simulink model "OCC_DQ_RCC_PO_BOOST_COMMON_GROUND_UPM"  (R2023a)
settings: Solver=ode1  StartTime=0.0  StopTime=5  FixedStep=1e-6  MaxStep=1e-6  RelTol=1e-3  EnableMultiTasking=on
undefined symbols (not defined in the file or in its folder): DiscIntNeverNeededParam
libraries: simulink x15, spsSeriesRLCBranchLib x14, spsVoltageMeasurementLib x8, slpidlib x7, spsDiodeLib x6, spsFirstOrderFilterLib x6, spsMosfetLib x5, powerlib_extras x5, spsCurrentMeasurementLib x4, spsAlphaBetaZerotodq0Lib x3, eePowerMeasurement x2, spsACVoltageSourceLib x1
(part 2 of 2)

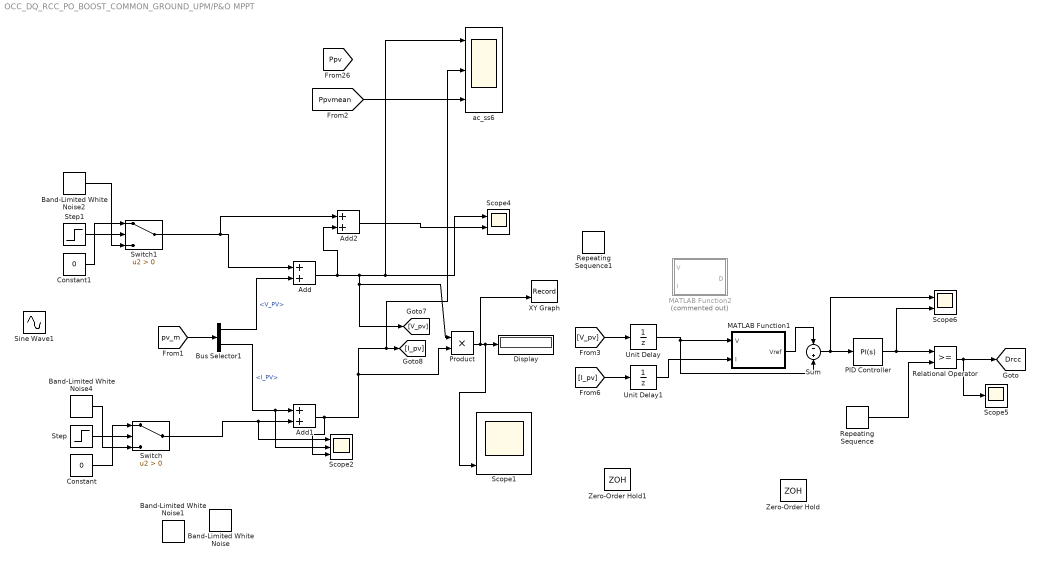
== system OCC_DQ_RCC_PO_BOOST_COMMON_GROUND_UPM/P&O MPPT  ==
  Add : Sum
  Add1 : Sum
  Add2 : Sum
  Band-Limited White Noise : simulink/Sources/Band-Limited White Noise  Cov=[1.74e-6]  Ts=1e-6  seed=[23341]
  Band-Limited White Noise1 : simulink/Sources/Band-Limited White Noise  Cov=[5.776e-9]  Ts=1e-6  seed=[23341]
  Band-Limited White Noise2 : simulink/Sources/Band-Limited White Noise  Cov=[6.6e-7]  Ts=1e-6  seed=[23341]
  Band-Limited White Noise4 : simulink/Sources/Band-Limited White Noise  Cov=[3.58e-10]  Ts=1e-6  seed=[23341]
  Bus Selector1 : BusSelector  OutputSignals=V_PV,I_PV
  Constant : Constant  Value=0
  Constant1 : Constant  Value=0
  Display : Display
  MATLAB Function1 : MATLAB Function  TreatAsAtomicUnit=on
  MATLAB Function2 : MATLAB Function  Commented=on  TreatAsAtomicUnit=on
  PID Controller : slpidlib/PID Controller  Controller=PI  Form=Parallel  TimeDomain=Continuous-time  UseExternalTs=off  SampleTime=-1  IntegratorMethod=Forward Euler  FilterMethod=Forward Euler  ControllerParametersSource=internal  P=0.011  I=15  UseKiTs=off  D=0  N=100  UseFilter=on  TunerSelectOption=Transfer Function Based (PID Tuner App)  InitialConditionSource=internal  InitialConditionForIntegrator=0  InitialConditionForFilter=0  DifferentiatorICPrevScaledInput=0  ExternalReset=none  TrackingMode=off  Kt=1  LimitOutput=on  SatLimitsSource=internal  UpperSaturationLimit=0.95  LowerSaturationLimit=0  LinearizeAsGain=on  AntiWindupMode=none  Kb=1  LimitIntegrator=off  UpperIntegratorSaturationLimit=inf  LowerIntegratorSaturationLimit=-inf  POutMin=[]  POutMax=[]  IOutMin=[]  IOutMax=[]  DOutMin=[]  DOutMax=[]  NOutMin=[]  NOutMax=[]  SumOutMin=[]  SumOutMax=[]  SaturationOutMin=[]  SaturationOutMax=[]  PParamMin=[]  PParamMax=[]  IParamMin=[]  IParamMax=[]  DParamMin=[]  DParamMax=[]  NParamMin=[]  NParamMax=[]  KbParamMin=[]  KbParamMax=[]  KtParamMin=[]  KtParamMax=[]  KbOutMin=[]  KbOutMax=[]  KtOutMin=[]  KtOutMax=[]  IntegratorOutMin=[]  IntegratorOutMax=[]  FilterOutMin=[]  FilterOutMax=[]  SumI1OutMin=[]  SumI1OutMax=[]  SumI2OutMin=[]  SumI2OutMax=[]  SumI3OutMin=[]  SumI3OutMax=[]  SumI4OutMin=[]  SumI4OutMax=[]  SumDOutMin=[]  SumDOutMax=[]  DifferentiatorOutMin=[]  DifferentiatorOutMax=[]  FilterDiffOutCoefMin=[]  FilterDiffOutCoefMax=[]  ReciprocalOutMin=[]  ReciprocalOutMax=[]  SumDenOutMin=[]  SumDenOutMax=[]  SumNumOutMin=[]  SumNumOutMax=[]  DivideOutMin=[]  DivideOutMax=[]  UdiffTsProdOutMin=[]  UdiffTsProdOutMax=[]  NTsProdOutMin=[]  NTsProdOutMax=[]  UintegralTsProdOutMin=[]  UintegralTsProdOutMax=[]  UngainTsProdOutMin=[]  UngainTsProdOutMax=[]  ClampingZeroOutDataTypeStr=Inherit: Inherit via back propagation  ClampingZeroOutMin=[]  ClampingZeroOutMax=[]  FilterDenConstantOutDataTypeStr=Inherit: Inherit via back propagation  FilterDenConstantOutMin=[]  FilterDenConstantOutMax=[]  PCopyOutDataTypeStr=Inherit: Inherit via back propagation  PCopyOutMin=[]  PCopyOutMax=[]  NCopyOutDataTypeStr=Inherit: Inherit via back propagation  NCopyOutMin=[]  NCopyOutMax=[]  IntegratorContinuousStateAttributes=''  IntegratorStateMustResolveToSignalObject=off  IntegratorRTWStateStorageClass=Auto  FilterContinuousStateAttributes=''  FilterStateMustResolveToSignalObject=off  FilterRTWStateStorageClass=Auto  ParallelPVariant=InternalParameters  IdealPVariant=Disabled  IVariant=InternalParameters  DVariant=Disabled  IntegratorVariant=Continuous  SatVariant=Enabled  AWVariant=Passthrough  PCopyVariant=Disabled  TRVariant=Disabled  FdbkBlocksVariant=Forward  IdealPFdbkVariant=Disabled  SatFdbkVariant=Disabled  DerivativeFilterVariant=Disabled  NVariant=Disabled  NCopyVariant=Disabled_SignalSpec  FilterICVariant=Disabled  IntegratorICVariant=InternalICs  ExternalResetVariant=Disabled  TRSumVariant=Passthrough  SumFdbkVariant=Disabled  SumVariant=Sum_PI  TsampFilterVariant=InternalTs  TsampNgainVariant=Passthrough  TsampIntegralVariant=Disabled_SignalSpec  ExternalSaturationOutDataTypeStr=Inherit: Same as second input
  Product : Product
  Relational Operator : RelationalOperator  OutDataTypeStr=boolean  RndMeth=Simplest  InputSameDT=off
  Repeating Sequence : simulink/Sources/Repeating Sequence  rep_seq_t=[0 5e-5 1e-4]  rep_seq_y=[0 1 0]
  Repeating Sequence1 : simulink/Sources/Repeating Sequence  rep_seq_t=[0 2]  rep_seq_y=[0 2]
  Scope1 : Scope  NumInputPorts=3
  Scope2 : Scope  NumInputPorts=3
  Scope4 : Scope  NumInputPorts=2
  Scope5 : Scope
  Scope6 : Scope  NumInputPorts=2
  Sine Wave1 : Sin  Amplitude=0.5  Frequency=80000*pi  SampleTime=0
  Step : Step  Time=4  SampleTime=0
  Step1 : Step  Time=4  SampleTime=0
  Sum : Sum  Inputs=-+
  Switch : Switch  Criteria=u2 > Threshold  SaturateOnIntegerOverflow=off  InputSameDT=off
  Switch1 : Switch  Criteria=u2 > Threshold  SaturateOnIntegerOverflow=off  InputSameDT=off
  Unit Delay : UnitDelay  SampleTime=1e-6  HasFrameUpgradeWarning=on
  Unit Delay1 : UnitDelay  SampleTime=1e-6  HasFrameUpgradeWarning=on
  XY Graph : Record  FileSettingsInternal="{\"entries\":[{\"content\":{\"excelSettings\":{\"content\":{},\"type\":\"Streamout.ExcelSettings\"}},\"type\":\"Streamout.FileSettingStorage\",\"uuid\":\"\"}],\"packageUris\":[\"http:\\/\\/schema.mathworks.com\\/mf0\\/streamout_blocks\\/R2020a\"],\"version\":\"1.0\"}"  Layout=[1 1]  SignalsInternal="{\"entries\":[{\"content\":{},\"type\":\"RecordBlkView.InputSignals\",\"uuid\":\"\"}],\"packageUris\":[\"http:\\/\\/schema.mathworks.com\\/mf0\\/streamout_blocks\\/R2020a\"],\"version\":\"1.0\"}"  CompatibilityTag=XY
  Zero-Order Hold : ZeroOrderHold  SampleTime=-1
  Zero-Order Hold1 : ZeroOrderHold  SampleTime=-1
  ac_ss6 : Scope  NumInputPorts=3
  tag scope: Drcc=global
  wires:
  [I_pv] -> Unit Delay1/1
  Unit Delay/1 -> MATLAB Function1/1(V), Sum/2
  Relational Operator/1 -> [Drcc], Scope5/1
  Repeating Sequence/1 -> Relational Operator/2
  Unit Delay1/1 -> MATLAB Function1/2(I)
  PID Controller/1 -> Scope6/2, Relational Operator/1
  Product/1 -> XY Graph/2, Scope1/3, Display/1
  MATLAB Function1/1(Vref) -> Sum/1
  Sum/1 -> Scope6/1, PID Controller/1
  [V_pv] -> Unit Delay/1
  Bus Selector1/2 -> Scope2/2, Add1/1  "<I_PV>"
  [pv_m] -> Bus Selector1/1
  Bus Selector1/1 -> Add/2  "<V_PV>"
  Switch1/1 -> Add2/1, Add/1
  Add2/1 -> Scope4/2
  Band-Limited White Noise2/1 -> Switch1/3
  Step1/1 -> Switch1/2
  Constant1/1 -> Switch1/1
  Switch/1 -> Scope2/1, Add1/2
  Step/1 -> Switch/2
  Constant/1 -> Switch/1
  Band-Limited White Noise4/1 -> Switch/3
  Add1/1 -> Scope2/3, Product/2, ac_ss6/2, [I_pv]
  Add/1 -> Add2/2, ac_ss6/1, Scope4/1, Product/1, [V_pv]
  [Ppvmean] -> ac_ss6/3

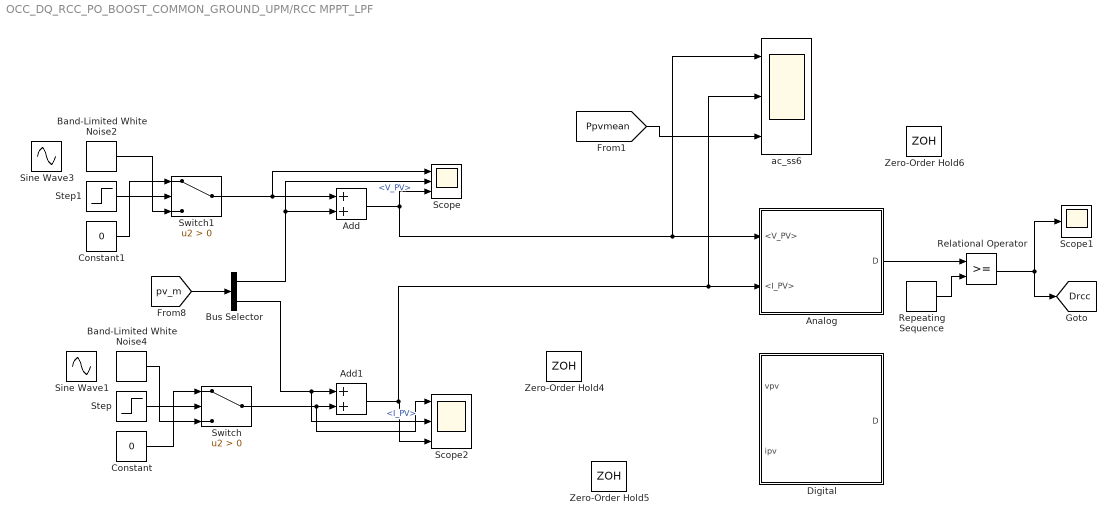
== system OCC_DQ_RCC_PO_BOOST_COMMON_GROUND_UPM/RCC MPPT_LPF ==
  Add : Sum
  Add1 : Sum
  Analog : Subsystem
  Band-Limited White Noise2 : simulink/Sources/Band-Limited White Noise  Cov=[6.6e-7]  Ts=1e-6  seed=[23341]
  Band-Limited White Noise4 : simulink/Sources/Band-Limited White Noise  Cov=[3.58e-10]  Ts=1e-6  seed=[23341]
  Bus Selector : BusSelector  OutputSignals=V_PV,I_PV
  Constant : Constant  Value=0
  Constant1 : Constant  Value=0
  Digital : Subsystem
  Relational Operator : RelationalOperator  OutDataTypeStr=boolean  RndMeth=Simplest  InputSameDT=off
  Repeating Sequence : simulink/Sources/Repeating Sequence  rep_seq_t=[0 5e-5 1e-4]  rep_seq_y=[0 1 0]
  Scope : Scope  NumInputPorts=3
  Scope1 : Scope
  Scope2 : Scope  NumInputPorts=3
  Sine Wave1 : Sin  Amplitude=0.1  Frequency=5*100000*pi  SampleTime=0
  Sine Wave3 : Sin  Frequency=5*100000*pi  SampleTime=0
  Step : Step  Time=4  SampleTime=0
  Step1 : Step  Time=4  SampleTime=0
  Switch : Switch  Criteria=u2 > Threshold  SaturateOnIntegerOverflow=off  InputSameDT=off
  Switch1 : Switch  Criteria=u2 > Threshold  SaturateOnIntegerOverflow=off  InputSameDT=off
  Zero-Order Hold4 : ZeroOrderHold  SampleTime=1e-4
  Zero-Order Hold5 : ZeroOrderHold  SampleTime=1e-4
  Zero-Order Hold6 : ZeroOrderHold  SampleTime=1e-4
  ac_ss6 : Scope  NumInputPorts=3
  tag scope: Drcc=global
  wires:
  [pv_m] -> Bus Selector/1
  Repeating Sequence/1 -> Relational Operator/2
  Relational Operator/1 -> [Drcc], Scope1/1
  Bus Selector/1 -> Add/2, Scope/2  "<V_PV>"
  Bus Selector/2 -> Scope2/2, Add1/1  "<I_PV>"
  Switch1/1 -> Scope/1, Add/1
  Step/1 -> Switch/2
  Switch/1 -> Scope2/1, Add1/2
  Step1/1 -> Switch1/2
  Constant/1 -> Switch/1
  Band-Limited White Noise4/1 -> Switch/3
  Band-Limited White Noise2/1 -> Switch1/3
  Constant1/1 -> Switch1/1
  Add1/1 -> ac_ss6/2, Analog/2(<I_PV>), Scope2/3
  Add/1 -> ac_ss6/1, Analog/1(<V_PV>), Scope/3
  Analog/1(D) -> Relational Operator/1
  [Ppvmean] -> ac_ss6/3

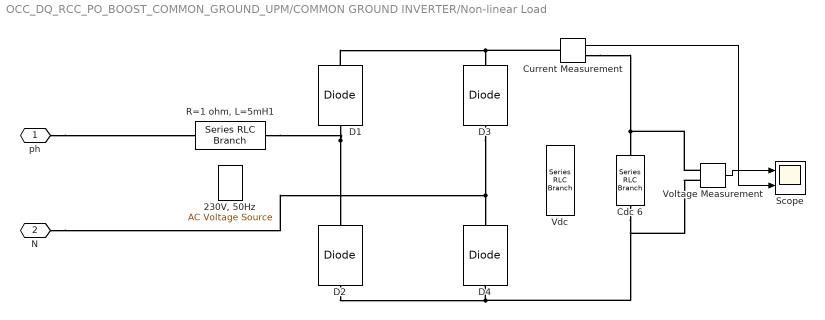
== system OCC_DQ_RCC_PO_BOOST_COMMON_GROUND_UPM/COMMON GROUND INVERTER/Non-linear Load ==
  "230V, 50Hz" : spsACVoltageSourceLib/AC Voltage Source  Amplitude=230*sqrt(2)  Phase=0  Frequency=50  SampleTime=0  Measurements=None  BusType=swing  Pref=10e3  Qref=0  Qmin=-inf  Qmax=+inf
  Cdc 6 : spsSeriesRLCBranchLib/Series RLC Branch  LConnTagsString=__new0  RConnTagsString=__new0  BranchType=RL  Resistance=8.57  Inductance=181e-3  SetiL0=off  InitialCurrent=0  Capacitance=2200e-6  Setx0=off  InitialVoltage=0  Measurements=Branch voltage and current
  Current Measurement : spsCurrentMeasurementLib/Current Measurement  PhasorSimulation=off  OutputType=Complex  PSBequivalent=0
  D{1..4} (4 alike) : spsDiodeLib/Diode  Ron=0.001  Lon=0  Vf=0.8  IC=0  UseSnubber=0  Rs=500  Cs=250e-9  Measurements=off
  "R=1 ohm, L=5mH1" : spsSeriesRLCBranchLib/Series RLC Branch  LConnTagsString=__new0  RConnTagsString=__new0  BranchType=L  Resistance=0.01  Inductance=5e-3  SetiL0=off  InitialCurrent=0  Capacitance=1e-6  Setx0=off  InitialVoltage=0  Measurements=Branch voltage and current
  Scope : Scope  NumInputPorts=2
  Vdc : spsSeriesRLCBranchLib/Series RLC Branch  LConnTagsString=__new0  RConnTagsString=__new0  BranchType=C  Resistance=1  Inductance=15.5e-3  SetiL0=off  InitialCurrent=0  Capacitance=10e-6  Setx0=off  InitialVoltage=0  Measurements=Branch voltage and current
  Voltage Measurement : spsVoltageMeasurementLib/Voltage Measurement  PhasorSimulation=off  OutputType=Complex  PSBequivalent=0
  ph : PMIOPort  Side=Left
  N : PMIOPort  Port=2  Side=Left
  wires:
  Voltage Measurement/1 -> Scope/1
  Current Measurement/1 -> Scope/2
  connections:
  D2/LConn1 -- Cdc 6/RConn1 -- Voltage Measurement/LConn2 -- D4/LConn1
  Voltage Measurement/LConn1 -- Current Measurement/RConn1 -- Cdc 6/LConn1
  D1/LConn1 -- "R=1 ohm, L=5mH1"/RConn1 -- D2/RConn1
  D3/LConn1 -- N/RConn1 -- D4/RConn1
  ph/RConn1 -- "R=1 ohm, L=5mH1"/LConn1
  D1/RConn1 -- Current Measurement/LConn1 -- D3/RConn1

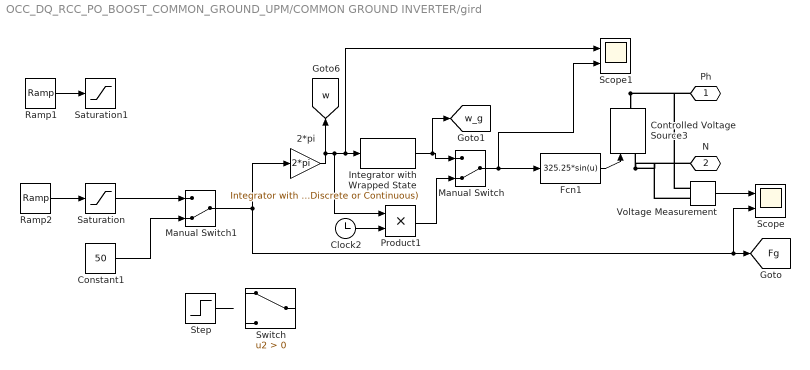
== system OCC_DQ_RCC_PO_BOOST_COMMON_GROUND_UPM/COMMON GROUND INVERTER/gird ==
  2*pi : Gain  Gain=2*pi
  Clock2 : Clock
  Constant1 : Constant  Value=50
  Controlled Voltage Source3 : spsControlledVoltageSourceLib/Controlled Voltage Source  Initialize=on  Source_Type=DC  Amplitude=0  Phase=0  Frequency=50  Measurements=None
  Fcn1 : Fcn  Expr=325.25*sin(u)
  Integrator with Wrapped State : eeGeneralControl/Integrator with Wrapped State (Discrete or Continuous)  LabelModeActiveChoice=Discrete  WrappedStateUpperValue=2*pi  WrappedStateLowerValue=0  x0=0  Ts=1e-5
      settings: LibrarySourceBlock=|
      | ee_sl_lib/General Control/Integrator with
      | Wrapped State
      | (Discrete or Continuous)
  Manual Switch : ManualSwitch  CurrentSetting=0
  Manual Switch1 : ManualSwitch  CurrentSetting=0
  Product1 : Product
  Ramp1 : simulink/Sources/Ramp  slope=2  start=1  InitialOutput=49.5
  Ramp2 : simulink/Sources/Ramp  slope=-2  start=1  InitialOutput=50
  Saturation : Saturate  UpperLimit=50  LowerLimit=49.5
  Saturation1 : Saturate  UpperLimit=50  LowerLimit=49.5
  Scope : Scope  NumInputPorts=2
  Scope1 : Scope  NumInputPorts=2
  Step : Step  After=0  SampleTime=0
  Switch : Switch  Criteria=u2 > Threshold  SaturateOnIntegerOverflow=off  InputSameDT=off
  Voltage Measurement : spsVoltageMeasurementLib/Voltage Measurement  PhasorSimulation=off  OutputType=Complex  PSBequivalent=0
  Ph : PMIOPort  Side=Left
  N : PMIOPort  Port=2  Side=Left
  tag scope: Fg=global, w=global, w_g=global
  wires:
  Voltage Measurement/1 -> Scope/1
  Ramp1/1 -> Saturation1/1
  Fcn1/1 -> Controlled Voltage Source3/1
  Clock2/1 -> Product1/2
  Integrator with Wrapped State/1 -> [w_g], Manual Switch/1
  Manual Switch/1 -> Fcn1/1, Scope1/2
  Product1/1 -> Manual Switch/2
  2*pi/1 -> Product1/1, Scope1/1, Integrator with Wrapped State/1, [w]
  Ramp2/1 -> Saturation/1
  Step/1 -> ?
  Constant1/1 -> Manual Switch1/2
  Saturation/1 -> Manual Switch1/1
  Manual Switch1/1 -> 2*pi/1, Scope/2, [Fg]
  connections:
  Controlled Voltage Source3/LConn1 -- Voltage Measurement/LConn2 -- N/RConn1
  Controlled Voltage Source3/RConn1 -- Voltage Measurement/LConn1 -- Ph/RConn1

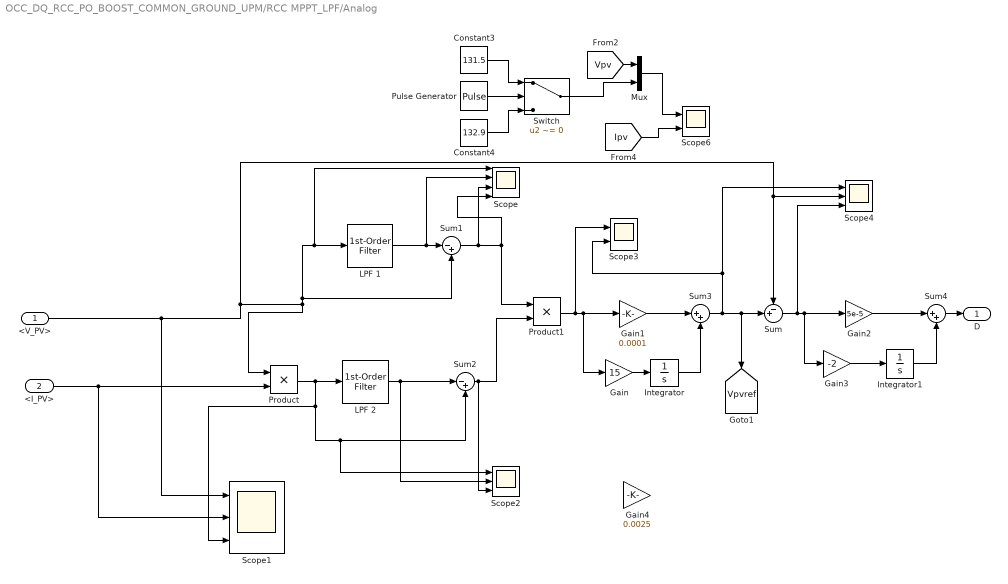
== system OCC_DQ_RCC_PO_BOOST_COMMON_GROUND_UPM/RCC MPPT_LPF/Analog ==
  <V_PV> : Inport
  <I_PV> : Inport  Port=2
  Constant3 : Constant  Value=131.5
  Constant4 : Constant  Value=132.9
  Gain : Gain  Gain=15
  Gain1 : Gain  Gain=0.0001
  Gain2 : Gain  Gain=5e-5
  Gain3 : Gain  Gain=-2
  Gain4 : Gain  Gain=0.0025
  Integrator : Integrator  InitialCondition=150  LimitOutput=on  UpperSaturationLimit=150  LowerSaturationLimit=100
  Integrator1 : Integrator  LimitOutput=on  UpperSaturationLimit=1  LowerSaturationLimit=-1
  LPF 1 : powerlib_extras/Control  Blocks/1st-Order  Filter  FilterType=Lowpass  Tc=2.5e-3  Initialize=on  Vac_Init=[132 0 100]  Vdc_Init=132  PlotResponse=off  param1=[0 500 1]
  LPF 2 : powerlib_extras/Control  Blocks/1st-Order  Filter  FilterType=Lowpass  Tc=2.5e-3  Initialize=on  Vac_Init=[132 0 100]  Vdc_Init=132  PlotResponse=off  param1=[0 500 1]
  Mux : Mux  Inputs=2
  Product : Product  RndMeth=Zero
  Product1 : Product  RndMeth=Zero
  Pulse Generator : DiscretePulseGenerator  PulseType=Time based  Period=2.5  PulseWidth=50
  Scope : Scope  NumInputPorts=4
  Scope1 : Scope  NumInputPorts=3
  Scope2 : Scope  NumInputPorts=3
  Scope3 : Scope  NumInputPorts=2
  Scope4 : Scope  NumInputPorts=3
  Scope6 : Scope  NumInputPorts=2
  Sum : Sum  Inputs=-+|
  Sum1 : Sum  Inputs=|-+
  Sum2 : Sum  Inputs=|-+
  Sum3 : Sum  Inputs=|++
  Sum4 : Sum  Inputs=|++
  Switch : Switch  Criteria=u2 ~= 0  SaturateOnIntegerOverflow=off  InputSameDT=off
  D : Outport
  tag scope: Vpvref=global
  wires:
  LPF 2/1 -> Sum2/1, Scope2/2
  Sum/1 -> Scope4/3, Gain3/1, Gain2/1
  <V_PV>/1 -> Scope1/1, Scope4/2, Sum/1, Scope/1, LPF 1/1, Sum1/2, Product/1
  Sum3/1 -> Scope3/2, Scope4/1, Sum/2, [Vpvref]
  Product1/1 -> Scope3/1, Gain/1, Gain1/1
  Integrator/1 -> Sum3/2
  Mux/1 -> Scope6/1
  Sum1/1 -> Product1/1, Scope/4, Scope/3
  Gain3/1 -> Integrator1/1
  Product/1 -> LPF 2/1, Scope1/3, Scope2/1, Sum2/2
  LPF 1/1 -> Scope/2, Sum1/1
  Integrator1/1 -> Sum4/2
  Constant4/1 -> Switch/3
  Switch/1 -> Mux/2
  Sum2/1 -> Product1/2, Scope2/3
  Gain/1 -> Integrator/1
  Constant3/1 -> Switch/1
  [Ipv] -> Scope6/2
  [Vpv] -> Mux/1
  Pulse Generator/1 -> Switch/2
  Gain2/1 -> Sum4/1
  Gain1/1 -> Sum3/1
  <I_PV>/1 -> Scope1/2, Product/2
  Sum4/1 -> D/1

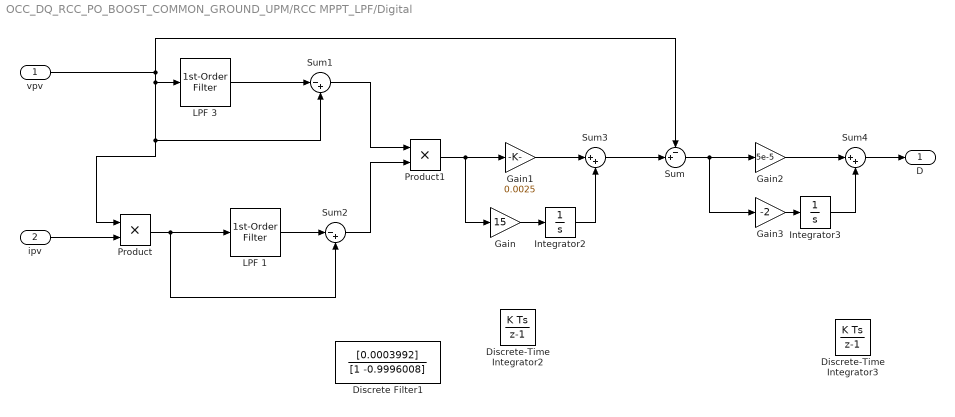
== system OCC_DQ_RCC_PO_BOOST_COMMON_GROUND_UPM/RCC MPPT_LPF/Digital ==
  vpv : Inport
  ipv : Inport  Port=2
  Discrete Filter1 : DiscreteFilter  Numerator=[0.0003992]  Denominator=[1 -0.9996008]
  Discrete-Time Integrator2 : DiscreteIntegrator  InitialCondition=180  SampleTime=1e-5  LimitOutput=on  UpperSaturationLimit=180  LowerSaturationLimit=100  ICPrevOutput=DiscIntNeverNeededParam  ICPrevScaledInput=DiscIntNeverNeededParam
  Discrete-Time Integrator3 : DiscreteIntegrator  SampleTime=1e-5  LimitOutput=on  UpperSaturationLimit=1  LowerSaturationLimit=-1  ICPrevOutput=DiscIntNeverNeededParam  ICPrevScaledInput=DiscIntNeverNeededParam
  Gain : Gain  Gain=15
  Gain1 : Gain  Gain=0.0025
  Gain2 : Gain  Gain=5e-5
  Gain3 : Gain  Gain=-2
  Integrator2 : Integrator  InitialCondition=150  LimitOutput=on  UpperSaturationLimit=180  LowerSaturationLimit=100
  Integrator3 : Integrator  LimitOutput=on  UpperSaturationLimit=1  LowerSaturationLimit=-1
  LPF 1 : powerlib_extras/Control  Blocks/1st-Order  Filter  FilterType=Lowpass  Tc=2.5e-3  Initialize=on  Vac_Init=[132 0 100]  Vdc_Init=132  PlotResponse=off  param1=[0 500 1]
  LPF 3 : powerlib_extras/Control  Blocks/1st-Order  Filter  FilterType=Lowpass  Tc=2.5e-3  Initialize=on  Vac_Init=[132 0 100]  Vdc_Init=132  PlotResponse=off  param1=[0 500 1]
  Product : Product  RndMeth=Zero
  Product1 : Product  RndMeth=Zero
  Sum : Sum  Inputs=-+|
  Sum1 : Sum  Inputs=|-+
  Sum2 : Sum  Inputs=|-+
  Sum3 : Sum  Inputs=|++
  Sum4 : Sum  Inputs=|++
  D : Outport
  wires:
  Gain2/1 -> Sum4/1
  Product1/1 -> Gain/1, Gain1/1
  vpv/1 -> Sum/1, LPF 3/1, Product/1, Sum1/2
  Sum3/1 -> Sum/2
  ipv/1 -> Product/2
  Sum4/1 -> D/1
  Gain1/1 -> Sum3/1
  Gain/1 -> Integrator2/1
  Sum1/1 -> Product1/1
  Gain3/1 -> Integrator3/1
  LPF 3/1 -> Sum1/1
  Integrator3/1 -> Sum4/2
  Product/1 -> Sum2/2, LPF 1/1
  Sum/1 -> Gain3/1, Gain2/1
  Integrator2/1 -> Sum3/2
  Sum2/1 -> Product1/2
  LPF 1/1 -> Sum2/1

== matlab function OCC_DQ_RCC_PO_BOOST_COMMON_GROUND_UPM/P&O MPPT /MATLAB Function1 ==
  data: V input; Vref output; I input
function Vref =RefGen(V,I)
Vrefmax=32.9*5;% Voc
Vrefmin = 0;
Vrefinit = 26.3*5;%aprrox mmp voltage
deltaVref=0.00000025;
persistent Vold Pold Vrefold;
dataType = 'double';


if isempty (Vold)
Vold=0;
Pold=0;
Vrefold=Vrefinit;
end
P=V*I;
dV=V-Vold;
dP=P-Pold;
if dP==0
    if dP<0
        if dV<0
        Vref=Vrefold+deltaVref;
        else 
            Vref= Vrefold-deltaVref;
        end
    else
        if dV<0
        Vref=Vrefold-deltaVref;
        else
            Vref = Vrefold+deltaVref;
         end
    end

else 
    Vref=Vrefold;
end
if  Vref>=Vrefmax|| Vref<=Vrefmin
    Vref = Vrefold;
end
Vrefold=Vref;
Vold= V;
Pold=P;

== matlab function OCC_DQ_RCC_PO_BOOST_COMMON_GROUND_UPM/P&O MPPT /MATLAB Function2 ==
  data: V input; D output; I input
% f =10000 hz (G)
function D  = PandO(V, I)
 
 
Dinit = 0.5;  %Initial value for D output
Dmax = 0.8;   %Maximum value for D
Dmin = 0.1;   %Minimum value for D
deltaD = 0.01; %Increment value used to increase/decrease the duty cycle D
 
 
persistent Vold Pold Dold;
 
dataType = 'double';
 
if isempty(Vold)
    Vold=0;
    Pold=0;
    Dold=Dinit;
end
P= V*I;
dV= V - Vold;
dP= P - Pold;
 
if dP ~= 0
    if dP < 0
        if dV < 0
            D = Dold - deltaD;
        else
            D = Dold + deltaD;
        end
    else
        if dV < 0
            D = Dold + deltaD;
        else
            D = Dold - deltaD;
        end    
    end
else
    D=Dold;
end
 
if D >= Dmax || D<= Dmin
    D=Dold;
end
 
Dold=D;
Vold=V;
Pold=P;

== matlab function OCC_DQ_RCC_PO_BOOST_COMMON_GROUND_UPM/DQ_CONTROL/MATLAB Function ==
  data: alpha input; y output; beta input
function y = fcn(alpha, beta)

y = sqrt(2*(alpha^2+beta^2));
